simulink model "NEPTUN_ZH_Z4"  (R2026a)
settings: Solver=VariableStepAuto  StopTime=20e-3  MaxStep=(185e-6)/25
libraries: simulink_extras x1
settings Model: Creator=Szalay  LastModifiedBy=Szalay

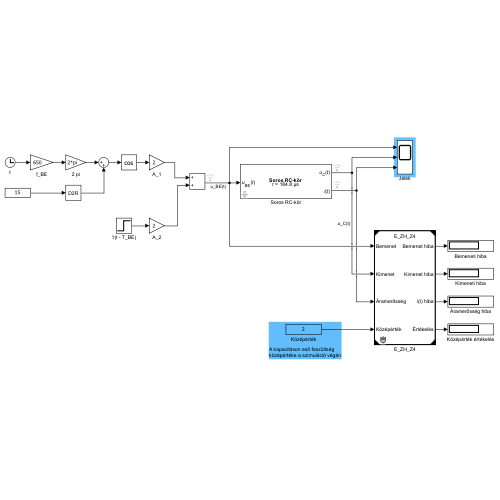
[thumbnail: Simulink's stored preview of the top-level diagram]
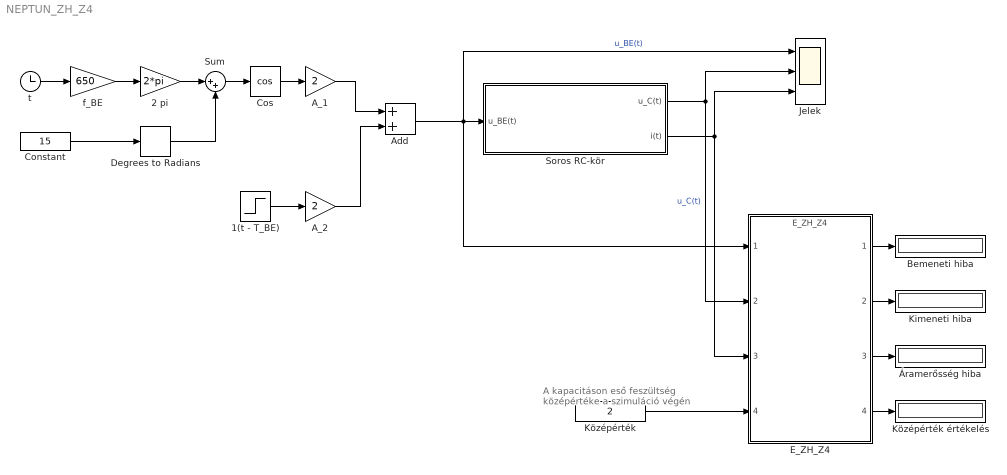
== system NEPTUN_ZH_Z4 ==
  note: A kapacitáson eső feszültség
      | középértéke a szimuláció végén
  1(t - T_BE) : Step  Time=10e-3  SampleTime=0
  2 pi : Gain  Gain=2*pi
  A_1 : Gain  Gain=2
  A_2 : Gain  Gain=2
  Add : Sum
  Bemeneti hiba : Display
  Constant : Constant  Value=15
  Cos : Trigonometry  Operator=cos
  Degrees to Radians : simulink_extras/Transformations/Degrees to Radians
  E_ZH_Z4 : ModelReference  ModelNameDialog=E_ZH_Z4.slxp  ModelReferenceVersion=3.5  CopyOfModelProtected=on
  Jelek : Scope  NumInputPorts=3
      settings: ActiveDisplayYMinimum=-1  ActiveDisplayYMaximum=1
  Kimeneti hiba : Display
  Középérték : Constant  Value=2
  Középérték értékelés : Display
  Soros RC-kör : Subsystem  mask(RC-kör){R=5600, C=33e-9, u_C0=2*cos(deg2rad(15)) - 5600*1e-3}
      mask prompts: R "Ellenállás"; C "Kapacitás"; u_C0 "Kezdeti kapacitás feszültség"
      mask help: A soros RC-kör modellje.
      mask DialogControl ParameterGroupVar Prompt: Modellparaméterek
      mask DialogControl Container3 Prompt: Kezdeti érték
      mask Display:
      | % Csatlakozók
      | port_label('input', 1, '{\itu}_{BE}({\itt})', 'texmode', 'on');
      | port_label('output', 1, '{\itu}_{\itC}({\itt})', 'texmode', 'on');
      | port_label('output', 2, '{\iti}({\itt})', 'texmode', 'on');
      | 
      | 
      | % Időállandó
      | R = str2double(get_param(gcb, 'R'));
      | C = str2double(get_param(gcb, 'C'));
      | 
      | tau = R*C;
      | 
      | % Felirat
      | text(0.5, 0.5, [ ...
      |     '{\bfSoros RC-kör}', newline, '{\it\tau} = ', ...
      |     sprintf('%g', 1e6*tau), ' \mus' ...
      |     ], ...
      |     'HorizontalAlignment', 'center', 'Interpreter', 'tex' ...
      |     );
  Sum : Sum  Inputs=|++
  f_BE : Gain  Gain=650
  t : Clock
  Áramerősség hiba : Display
  wires:
  Középérték/1 -> E_ZH_Z4/4
  E_ZH_Z4/4 -> Középérték értékelés/1
  E_ZH_Z4/2 -> Kimeneti hiba/1
  E_ZH_Z4/1 -> Bemeneti hiba/1
  E_ZH_Z4/3 -> Áramerősség hiba/1
  Add/1 -> E_ZH_Z4/1, Soros RC-kör/1(u_BE(t)), Jelek/1  "u_BE(t)"
  A_1/1 -> Add/1
  Cos/1 -> A_1/1
  Sum/1 -> Cos/1
  2 pi/1 -> Sum/1
  f_BE/1 -> 2 pi/1
  t/1 -> f_BE/1
  Constant/1 -> Degrees to Radians/1
  Degrees to Radians/1 -> Sum/2
  1(t - T_BE)/1 -> A_2/1
  A_2/1 -> Add/2
  Soros RC-kör/1(u_C(t)) -> E_ZH_Z4/2, Jelek/2  "u_C(t)"
  Soros RC-kör/2(i(t)) -> E_ZH_Z4/3, Jelek/3

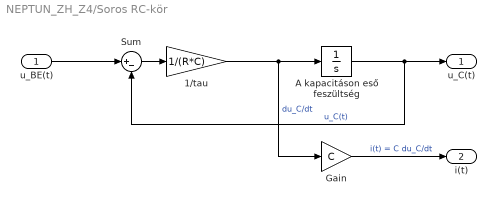
== system NEPTUN_ZH_Z4/Soros RC-kör ==
  u_BE(t) : Inport
  1/tau : Gain  Gain=1/(R*C)
  A kapacitáson eső feszültség : Integrator  InitialCondition=u_C0
  Gain : Gain  Gain=C
  Sum : Sum  Inputs=|+-
  u_C(t) : Outport
  i(t) : Outport  Port=2
  wires:
  1/tau/1 -> Gain/1, A kapacitáson eső feszültség/1  "du_C/dt"
  u_BE(t)/1 -> Sum/1
  Sum/1 -> 1/tau/1
  A kapacitáson eső feszültség/1 -> u_C(t)/1, Sum/2  "u_C(t)"
  Gain/1 -> i(t)/1  "i(t) = C du_C/dt"
